simulink model "Mot_Cooling_Model"  (R2026a)
settings: Solver=FixedStepAuto  StopTime=1372  FixedStep=1
values from neighbouring files (symbols this model uses):
  Cp_Coolant = 4182    [Motor_Cool.m]
  Cp_Mot = 1350    [Motor_Cool.m]
  Mass_flocoolant = Mot_CoolPow_Capability/(Cp_Coolant*(Temp_maxMHP-T_Amb))    [Motor_Cool.m]
  Mass_Mot = 23.69    [Motor_Cool.m]
  T_Amb = 18    [Motor_Cool.m]
  T_Mot_Intial = 20    [Motor_Cool.m]
settings Model: Creator=sujee  LastModifiedBy=sujee

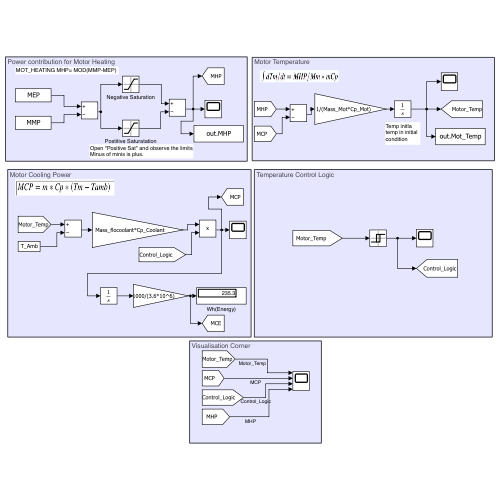
[thumbnail: Simulink's stored preview of the top-level diagram]
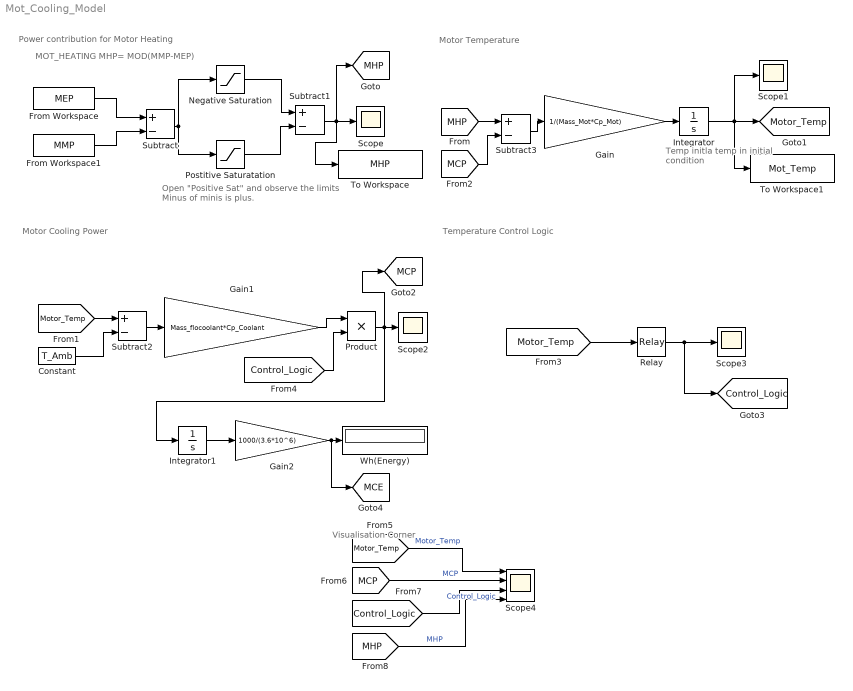
== system Mot_Cooling_Model ==
  note: Visualisation Corner
  note: Temperature Control Logic
  note: Motor Temperature
  note: Temp initla temp in initial condition
  note: Open "Positive Sat" and observe the limits
      | Minus of minis is plus.
  note: Power contribution for Motor Heating
  note: MOT_HEATING MHP= MOD(MMP-MEP)
  note: Motor Cooling Power
  Constant : Constant  Value=T_Amb
  From Workspace : FromWorkspace  VariableName=MEP
  From Workspace1 : FromWorkspace  VariableName=MMP
  Gain : Gain  Gain=1/(Mass_Mot*Cp_Mot)
  Gain1 : Gain  Gain=Mass_flocoolant*Cp_Coolant
  Gain2 : Gain  Gain=1000/(3.6*10^6)
  Integrator : Integrator  InitialCondition=T_Mot_Intial
  Integrator1 : Integrator
  Negative Saturation : Saturate  UpperLimit=inf  LowerLimit=0
  Postitive Saturatation : Saturate  UpperLimit=0  LowerLimit=-inf
  Product : Product
  Relay : Relay  OnSwitchValue=30  OffSwitchValue=20
  Scope{,1..3} (4 alike) : Scope
      Scope settings: ActiveDisplayYMinimum=-685.78882339305017  ActiveDisplayYMaximum=6172.0994105374521
      Scope1 settings: ActiveDisplayYMinimum=17.497464485252905  ActiveDisplayYMaximum=42.522819632723873
      Scope2 settings: ActiveDisplayYMinimum=-1  ActiveDisplayYMaximum=1  DataLoggingVariableName=ScopeData2
      Scope3 settings: ActiveDisplayYMinimum=-0.12499999999999997  ActiveDisplayYMaximum=1.125  DataLoggingVariableName=ScopeData3
  Scope4 : Scope  NumInputPorts=4
      settings: ActiveDisplayYMinimum=-1  ActiveDisplayYMaximum=1  DataLoggingVariableName=ScopeData4
  Subtract{,1..3} (4 alike) : Sum  Inputs=+-
  To Workspace : ToWorkspace  VariableName=MHP  SaveFormat=Timeseries  SampleTime=-1
  To Workspace1 : ToWorkspace  VariableName=Mot_Temp  SaveFormat=Timeseries  SampleTime=-1
  Wh(Energy) : Display
  tag scope: Control_Logic=global, MCE=global, MCP=global, MHP=global, Motor_Temp=global
  wires:
  From Workspace/1 -> Subtract/1
  From Workspace1/1 -> Subtract/2
  Subtract/1 -> Postitive Saturatation/1, Negative Saturation/1
  Subtract1/1 -> To Workspace/1, [MHP], Scope/1
  Negative Saturation/1 -> Subtract1/1
  Postitive Saturatation/1 -> Subtract1/2
  Gain/1 -> Integrator/1
  Integrator/1 -> To Workspace1/1, [Motor_Temp], Scope1/1
  [Motor_Temp] -> Subtract2/1
  Constant/1 -> Subtract2/2
  Subtract2/1 -> Gain1/1
  Gain1/1 -> Product/1
  [MHP] -> Subtract3/1
  Subtract3/1 -> Gain/1
  [MCP] -> Subtract3/2
  [Motor_Temp] -> Relay/1
  Relay/1 -> [Control_Logic], Scope3/1
  [Control_Logic] -> Product/2
  Product/1 -> Integrator1/1, [MCP], Scope2/1
  [Motor_Temp] -> Scope4/1  "Motor_Temp"
  [MCP] -> Scope4/2  "MCP"
  [Control_Logic] -> Scope4/3  "Control_Logic"
  [MHP] -> Scope4/4  "MHP"
  Integrator1/1 -> Gain2/1
  Gain2/1 -> [MCE], Wh(Energy)/1
